simulink model "tav1"  (R2025b)
settings: Solver=FixedStepAuto  StartTime=0.0  StopTime=20  FixedStep=0.005  RelTol=1e-3
libraries: robotmaniplib x12
settings Model: Creator=giuli  LastModifiedBy=Andrea

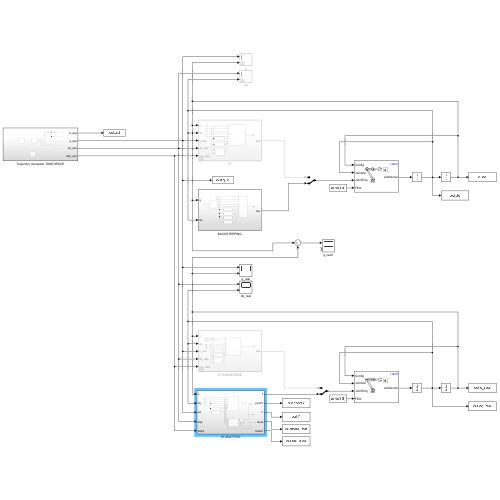
[thumbnail: Simulink's stored preview of the top-level diagram]
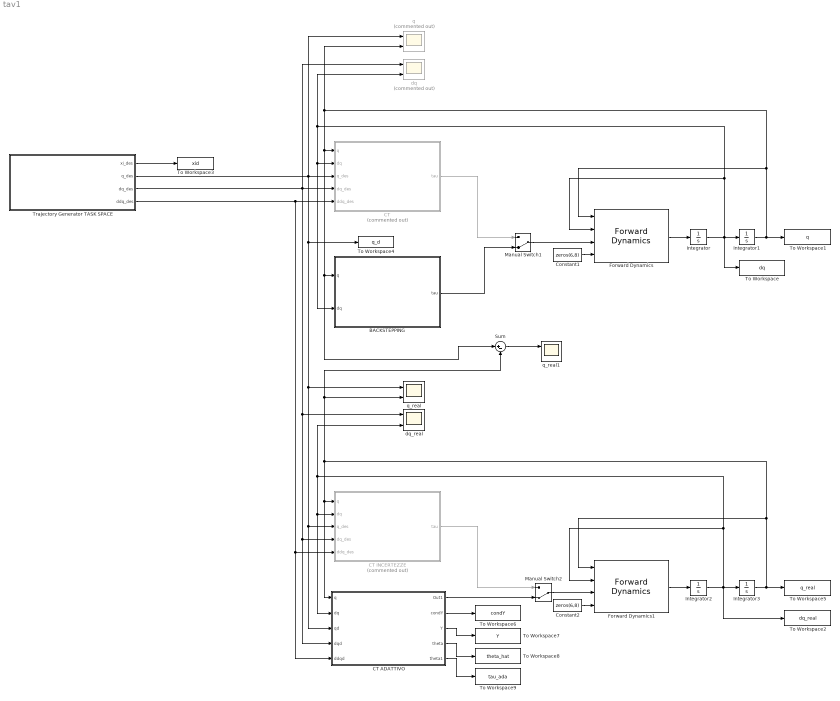
== system tav1 ==
  BACKSTEPPING : Subsystem
  CT : Subsystem  Commented=on
  CT ADATTIVO : Subsystem
  CT INCERTEZZE : Subsystem  Commented=on
  Constant1 : Constant  Value=zeros(6,8)
  Constant2 : Constant  Value=zeros(6,8)
  Forward Dynamics : robotmaniplib/Forward Dynamics  RigidBodyTree=robot  SimulateUsing=Interpreted execution
  Forward Dynamics1 : robotmaniplib/Forward Dynamics  RigidBodyTree=robot  SimulateUsing=Interpreted execution
  Integrator{,1..3} (4 alike) : Integrator  InitialCondition=zeros(6,1)
  Manual Switch1 : ManualSwitch  CurrentSetting=0
  Manual Switch2 : ManualSwitch  CurrentSetting=0
  Sum : Sum  Inputs=|+-
  To Workspace : ToWorkspace  VariableName=dq  SaveFormat=Timeseries  SampleTime=-1
  To Workspace1 : ToWorkspace  VariableName=q  SaveFormat=Timeseries  SampleTime=-1
  To Workspace2 : ToWorkspace  VariableName=dq_real  SaveFormat=Timeseries  SampleTime=-1
  To Workspace3 : ToWorkspace  VariableName=xid  SaveFormat=Timeseries  SampleTime=-1
  To Workspace4 : ToWorkspace  VariableName=q_d  SaveFormat=Timeseries  SampleTime=-1
  To Workspace5 : ToWorkspace  VariableName=q_real  SaveFormat=Timeseries  SampleTime=-1
  To Workspace6 : ToWorkspace  VariableName=condY  SaveFormat=Timeseries  SampleTime=-1
  To Workspace7 : ToWorkspace  VariableName=Y  SaveFormat=Timeseries  SampleTime=-1
  To Workspace8 : ToWorkspace  VariableName=theta_hat  SaveFormat=Timeseries  SampleTime=-1
  To Workspace9 : ToWorkspace  VariableName=tau_ada  SaveFormat=Timeseries  SampleTime=-1
  Trajectory Generator TASK SPACE : Subsystem
  dq : Scope  Commented=on  NumInputPorts=2
      settings: ActiveDisplayYMinimum=-3.470657788298241  ActiveDisplayYMaximum=1.9321669789401574  DataLoggingVariableName=ScopeData3
  dq_real : Scope  NumInputPorts=2
      settings: ActiveDisplayYMinimum=-6.9956803781599319  ActiveDisplayYMaximum=9.2235365390379016  DataLoggingVariableName=ScopeData2
  q : Scope  Commented=on  NumInputPorts=2
      settings: ActiveDisplayYMinimum=-2.5892485172575581  ActiveDisplayYMaximum=1.7379165019175062
  q_real : Scope  NumInputPorts=2
      settings: ActiveDisplayYMinimum=-6.9462044965016778  ActiveDisplayYMaximum=2.2220227218335191  DataLoggingVariableName=ScopeData4
  q_real1 : Scope  NumInputPorts=2
      settings: ActiveDisplayYMinimum=-0.19703612887750396  ActiveDisplayYMaximum=0.21289982446826508  DataLoggingVariableName=ScopeData5
  wires:
  Forward Dynamics/1 -> Integrator/1
  Integrator/1 -> To Workspace/1, Forward Dynamics/2, dq/2, BACKSTEPPING/2(dq), CT/2(dq), Integrator1/1
  Integrator1/1 -> q/2, Sum/1, BACKSTEPPING/1(q), CT/1(q), Forward Dynamics/1, To Workspace1/1
  Constant1/1 -> Forward Dynamics/4
  Trajectory Generator TASK SPACE/1(xi_des) -> To Workspace3/1
  Manual Switch1/1 -> Forward Dynamics/3
  CT/1(tau) -> Manual Switch1/1
  BACKSTEPPING/1(tau) -> Manual Switch1/2
  CT INCERTEZZE/1(tau) -> Manual Switch2/1
  Integrator2/1 -> Integrator3/1, dq_real/2, CT INCERTEZZE/2(dq), CT ADATTIVO/2(dq), Forward Dynamics1/2, To Workspace2/1
  Constant2/1 -> Forward Dynamics1/4
  Sum/1 -> q_real1/1
  Trajectory Generator TASK SPACE/4(ddq_des) -> CT ADATTIVO/5(ddqd), CT INCERTEZZE/5(ddq_des), CT/5(ddq_des)
  Trajectory Generator TASK SPACE/2(q_des) -> q/1, CT/3(q_des), CT ADATTIVO/3(qd), CT INCERTEZZE/3(q_des), q_real/1, To Workspace4/1
  Trajectory Generator TASK SPACE/3(dq_des) -> dq/1, CT/4(dq_des), CT ADATTIVO/4(dqd), CT INCERTEZZE/4(dq_des), dq_real/1
  Forward Dynamics1/1 -> Integrator2/1
  Manual Switch2/1 -> Forward Dynamics1/3
  Integrator3/1 -> To Workspace5/1, q_real/2, Sum/2, CT ADATTIVO/1(q), CT INCERTEZZE/1(q), Forward Dynamics1/1
  CT ADATTIVO/1(Out1) -> Manual Switch2/2
  CT ADATTIVO/2(condY) -> To Workspace6/1
  CT ADATTIVO/3(Y) -> To Workspace7/1
  CT ADATTIVO/4(theta) -> To Workspace8/1
  CT ADATTIVO/5(theta1) -> To Workspace9/1

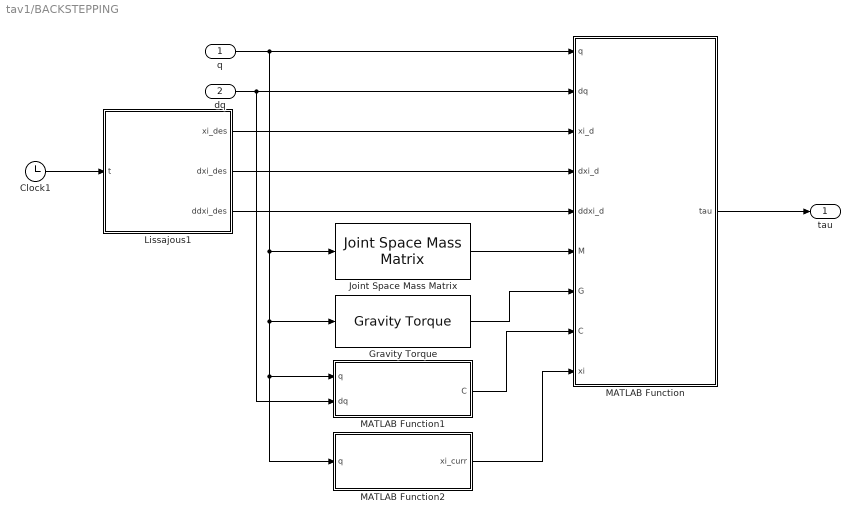
== system tav1/BACKSTEPPING ==
  q : Inport
  dq : Inport  Port=2
  Clock1 : Clock
  Gravity Torque : robotmaniplib/Gravity Torque  RigidBodyTree=robot  SimulateUsing=Interpreted execution
  Joint Space Mass Matrix : robotmaniplib/Joint Space Mass Matrix  RigidBodyTree=robot  SimulateUsing=Interpreted execution
  Lissajous1 : MATLAB Function  TreatAsAtomicUnit=on
  MATLAB Function : MATLAB Function  TreatAsAtomicUnit=on
  MATLAB Function1 : MATLAB Function  TreatAsAtomicUnit=on
  MATLAB Function2 : MATLAB Function  TreatAsAtomicUnit=on
  tau : Outport
  wires:
  dq/1 -> MATLAB Function1/2(dq), MATLAB Function/2(dq)
  q/1 -> Joint Space Mass Matrix/1, Gravity Torque/1, MATLAB Function2/1(q), MATLAB Function1/1(q), MATLAB Function/1(q)
  Joint Space Mass Matrix/1 -> MATLAB Function/6(M)
  Gravity Torque/1 -> MATLAB Function/7(G)
  MATLAB Function/1(tau) -> tau/1
  Clock1/1 -> Lissajous1/1(t)
  Lissajous1/1(xi_des) -> MATLAB Function/3(xi_d)
  Lissajous1/2(dxi_des) -> MATLAB Function/4(dxi_d)
  Lissajous1/3(ddxi_des) -> MATLAB Function/5(ddxi_d)
  MATLAB Function2/1(xi_curr) -> MATLAB Function/9(xi)
  MATLAB Function1/1(C) -> MATLAB Function/8(C)

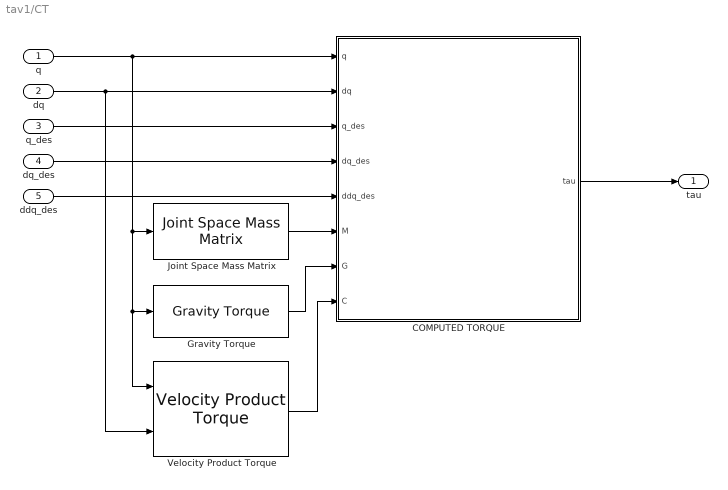
== system tav1/CT ==
  q : Inport
  dq : Inport  Port=2
  q_des : Inport  Port=3
  dq_des : Inport  Port=4
  ddq_des : Inport  Port=5
  COMPUTED TORQUE : MATLAB Function  TreatAsAtomicUnit=on
  Gravity Torque : robotmaniplib/Gravity Torque  RigidBodyTree=robot  SimulateUsing=Interpreted execution
  Joint Space Mass Matrix : robotmaniplib/Joint Space Mass Matrix  RigidBodyTree=robot  SimulateUsing=Interpreted execution
  Velocity Product Torque : robotmaniplib/Velocity Product Torque  RigidBodyTree=robot  SimulateUsing=Interpreted execution
  tau : Outport
  wires:
  COMPUTED TORQUE/1(tau) -> tau/1
  q_des/1 -> COMPUTED TORQUE/3(q_des)
  dq/1 -> Velocity Product Torque/2, COMPUTED TORQUE/2(dq)
  q/1 -> Velocity Product Torque/1, Gravity Torque/1, Joint Space Mass Matrix/1, COMPUTED TORQUE/1(q)
  dq_des/1 -> COMPUTED TORQUE/4(dq_des)
  ddq_des/1 -> COMPUTED TORQUE/5(ddq_des)
  Joint Space Mass Matrix/1 -> COMPUTED TORQUE/6(M)
  Gravity Torque/1 -> COMPUTED TORQUE/7(G)
  Velocity Product Torque/1 -> COMPUTED TORQUE/8(C)

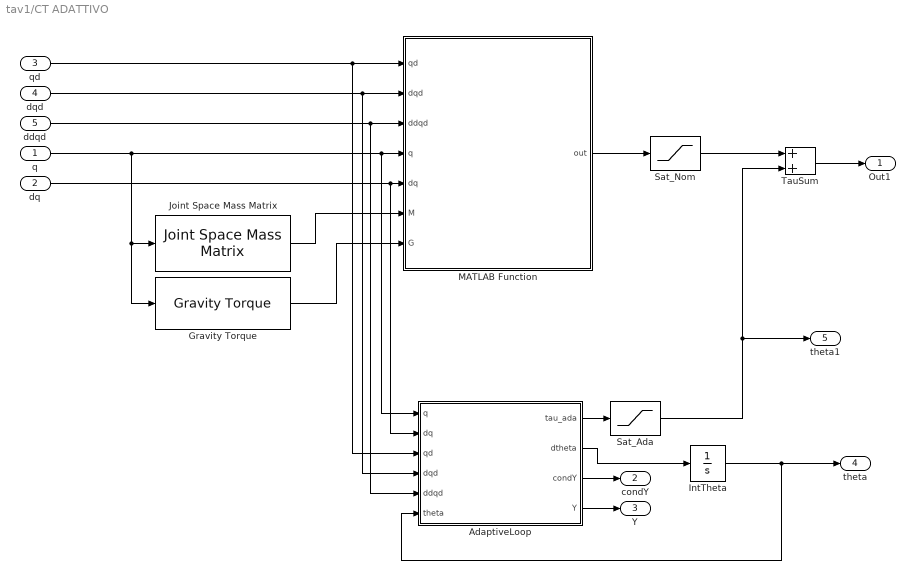
== system tav1/CT ADATTIVO ==
  q : Inport
  dq : Inport  Port=2
  qd : Inport  Port=3
  dqd : Inport  Port=4
  ddqd : Inport  Port=5
  AdaptiveLoop : MATLAB Function  TreatAsAtomicUnit=on
  Gravity Torque : robotmaniplib/Gravity Torque  RigidBodyTree=robot_real  SimulateUsing=Interpreted execution
  IntTheta : Integrator  InitialCondition=[0;0;0;0;0;0;0;0;0;0;0;0;0;0;0;0;0;0;0;0;0;0;0;0;0;0;0;0;0;0;0;0;0;0;0;0;0;0;0;0;0;0]
  Joint Space Mass Matrix : robotmaniplib/Joint Space Mass Matrix  RigidBodyTree=robot_real  SimulateUsing=Interpreted execution
  MATLAB Function : MATLAB Function  TreatAsAtomicUnit=on
  Sat_Ada : Saturate  UpperLimit=100  LowerLimit=-100
  Sat_Nom : Saturate  UpperLimit=100  LowerLimit=-100
  TauSum : Sum
  Out1 : Outport
  condY : Outport  Port=2
  Y : Outport  Port=3
  theta : Outport  Port=4
  theta1 : Outport  Port=5
  wires:
  q/1 -> AdaptiveLoop/1(q), MATLAB Function/4(q), Joint Space Mass Matrix/1, Gravity Torque/1
  Sat_Nom/1 -> TauSum/1
  qd/1 -> MATLAB Function/1(qd), AdaptiveLoop/3(qd)
  TauSum/1 -> Out1/1
  ddqd/1 -> MATLAB Function/3(ddqd), AdaptiveLoop/5(ddqd)
  AdaptiveLoop/1(tau_ada) -> Sat_Ada/1
  AdaptiveLoop/2(dtheta) -> IntTheta/1
  dq/1 -> AdaptiveLoop/2(dq), MATLAB Function/5(dq)
  Sat_Ada/1 -> TauSum/2, theta1/1
  IntTheta/1 -> theta/1, AdaptiveLoop/6(theta)
  dqd/1 -> MATLAB Function/2(dqd), AdaptiveLoop/4(dqd)
  MATLAB Function/1(out) -> Sat_Nom/1
  Gravity Torque/1 -> MATLAB Function/7(G)
  Joint Space Mass Matrix/1 -> MATLAB Function/6(M)
  AdaptiveLoop/3(condY) -> condY/1
  AdaptiveLoop/4(Y) -> Y/1

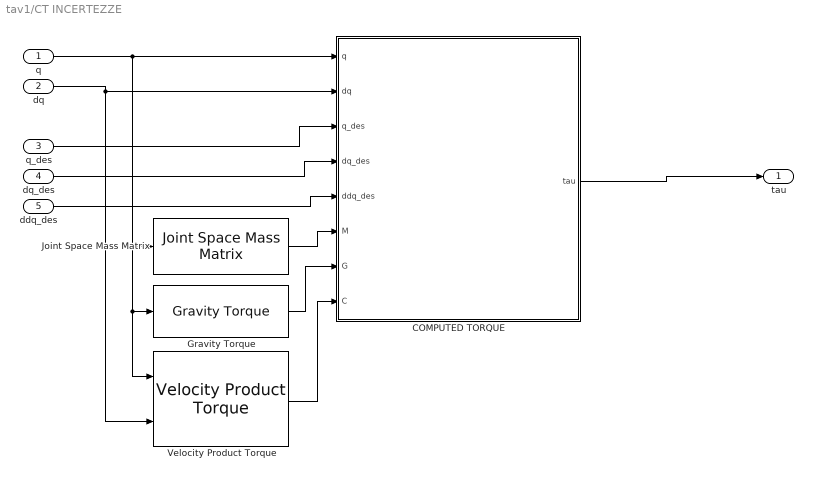
== system tav1/CT INCERTEZZE ==
  q : Inport
  dq : Inport  Port=2
  q_des : Inport  Port=3
  dq_des : Inport  Port=4
  ddq_des : Inport  Port=5
  COMPUTED TORQUE : MATLAB Function  TreatAsAtomicUnit=on
  Gravity Torque : robotmaniplib/Gravity Torque  RigidBodyTree=robot_real  SimulateUsing=Interpreted execution
  Joint Space Mass Matrix : robotmaniplib/Joint Space Mass Matrix  RigidBodyTree=robot_real  SimulateUsing=Interpreted execution
  Velocity Product Torque : robotmaniplib/Velocity Product Torque  RigidBodyTree=robot_real  SimulateUsing=Interpreted execution
  tau : Outport
  wires:
  COMPUTED TORQUE/1(tau) -> tau/1
  q_des/1 -> COMPUTED TORQUE/3(q_des)
  dq/1 -> Velocity Product Torque/2, COMPUTED TORQUE/2(dq)
  q/1 -> Velocity Product Torque/1, Gravity Torque/1, Joint Space Mass Matrix/1, COMPUTED TORQUE/1(q)
  dq_des/1 -> COMPUTED TORQUE/4(dq_des)
  ddq_des/1 -> COMPUTED TORQUE/5(ddq_des)
  Joint Space Mass Matrix/1 -> COMPUTED TORQUE/6(M)
  Gravity Torque/1 -> COMPUTED TORQUE/7(G)
  Velocity Product Torque/1 -> COMPUTED TORQUE/8(C)

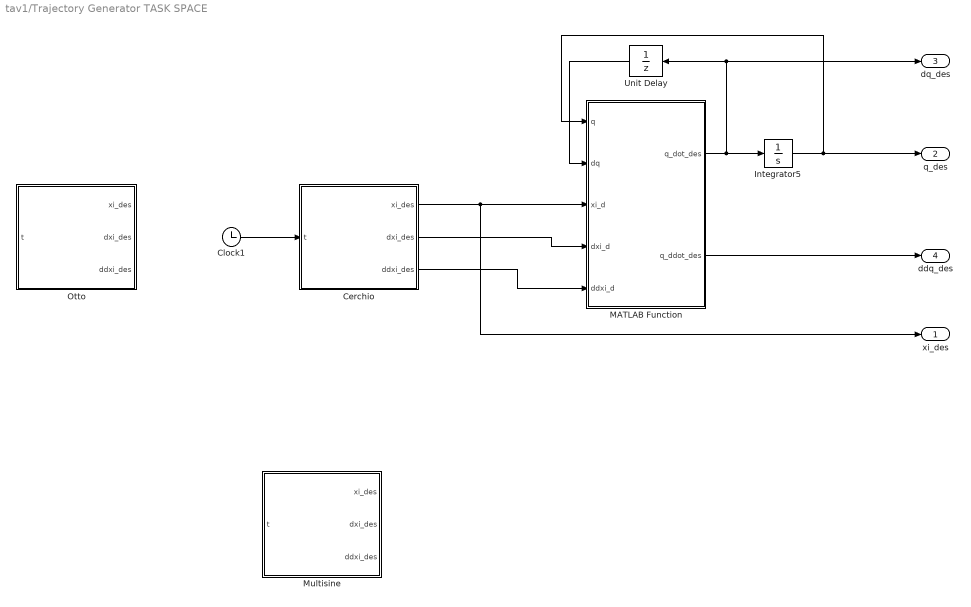
== system tav1/Trajectory Generator TASK SPACE ==
  Cerchio : MATLAB Function  TreatAsAtomicUnit=on
  Clock1 : Clock
  Integrator5 : Integrator  InitialCondition=[0;1.3052;-0.0773;-0;-1.2279;0]
  MATLAB Function : MATLAB Function  TreatAsAtomicUnit=on
  Multisine : MATLAB Function  TreatAsAtomicUnit=on
  Otto : MATLAB Function  TreatAsAtomicUnit=on
  Unit Delay : UnitDelay  InitialCondition=[0; 0.1; -0.073; 0; 0.2736; 0]  SampleTime=-1  HasFrameUpgradeWarning=on
  xi_des : Outport
  q_des : Outport  Port=2
  dq_des : Outport  Port=3
  ddq_des : Outport  Port=4
  wires:
  Unit Delay/1 -> MATLAB Function/2(dq)
  MATLAB Function/1(q_dot_des) -> Integrator5/1, Unit Delay/1, dq_des/1
  MATLAB Function/2(q_ddot_des) -> ddq_des/1
  Integrator5/1 -> q_des/1, MATLAB Function/1(q)
  Clock1/1 -> Cerchio/1(t)
  Cerchio/1(xi_des) -> xi_des/1, MATLAB Function/3(xi_d)
  Cerchio/2(dxi_des) -> MATLAB Function/4(dxi_d)
  Cerchio/3(ddxi_des) -> MATLAB Function/5(ddxi_d)

== matlab function tav1/CT INCERTEZZE/COMPUTED TORQUE ==
  data: q input; dq input; q_des input; dq_des input; ddq_des input; tau output; M input; G input; C input
function tau = computed_torque(q, dq, q_des, dq_des, ddq_des, M, G, C)

% control parameters
kp = 5;
kv = 2;

% error computation
e = q_des - q;
de = dq_des - dq;

tau = M*(ddq_des + kv*de + kp*e) + C + G;

== matlab function tav1/CT ADATTIVO/MATLAB Function ==
  data: qd input; out output; dqd input; ddqd input; q input; dq input; M input; G input
function out = fcn(qd,dqd,ddqd,q,dq, M, G)
    coder.extrinsic('velocityProduct');
    coder.extrinsic('evalin');
    
    % Recupero robot e nome end-effector dal base workspace
    robot = evalin('base','robot_real');                  % rigidBodyTree abbIrb120

    Kd   = 20*eye(6);
    Lam  = 2*eye(6);
    e    = qd-q;  de = dqd-dq;
    dqr  = ddqd + Lam*de;
    ar   = dqr  + Kd*(de+Lam*e);
    VP = zeros(6,1);  
    VP  = velocityProduct(robot, q, dq);   

    out = zeros(6,1);  
    out = M * ar + VP + G;

end

== matlab function tav1/Trajectory Generator TASK SPACE/Otto ==
  data: t input; xi_des output; dxi_des output; ddxi_des output
function [xi_des, dxi_des, ddxi_des] = traj_otto(t)
% FIGURA A OTTO (Lissajous 2:1)
%
% Punto iniziale IDENTICO al cerchio originale (lissajous.m):
%   t=0 -> xi = [0.50; 0.00; 0.10; 0; 0; 0]
%          dxi = [0; R*w; 0; 0; 0; 0] = [0; 0.30; 0; 0; 0; 0]
%
% Raccordo posizione:
%   x(t) = x0 + Rx * sin(2*w*t + pi/2)   →  x(0) = x0 + Rx = 0.50  ✓
%   y(t) = y0 + Ry * sin(w*t)             →  y(0) = 0               ✓
%   z(t) = z0                             →  z(0) = 0.10             ✓
%
% Raccordo velocità:
%   dx(0) = 2*w*Rx*cos(pi/2) = 0          ✓  (cerchio: dx(0) = 0)
%   dy(0) = w*Ry              = 0.30       →  Ry = 0.15 = R          ✓
%
% => Rx = Ry = R = 0.15, w = 2 (invariati dal cerchio)

%% Parametri (coerenti con lissajous.m)
x0 = 0.35;
y0 = 0.00;
z0 = 0.10;
R  = 0.15;
w  = 2.0;

%% Orientazione variabile (nulla a t=0, eccita Coriolis)
A_roll  = 0.10;   % ampiezza roll  [rad]
A_pitch = 0.08;   % ampiezza pitch [rad]
w_o     = 0.7;    % freq incommensurabile con w  → PE
% uso sin() → valore nullo a t=0  ✓

%% --- POSIZIONE ---
p_des = [ x0 + R * sin(2*w*t + pi/2);
          y0 + R * sin(w*t);
          z0                          ];

%% --- VELOCITÀ ---
dp_des = [ 2*w*R * cos(2*w*t + pi/2);
           w*R   * cos(w*t);
           0                          ];

%% --- ACCELERAZIONE ---
ddp_des = [ -4*w^2*R * sin(2*w*t + pi/2);
            -w^2*R   * sin(w*t);
             0                            ];

%% --- ORIENTAZIONE (sin -> 0 a t=0) ---
roll  = A_roll  * sin(w_o * t);
pitch = A_pitch * sin(w_o * t);
yaw   = 0;

o_des   = [roll; pitch; yaw];
do_des  = [ A_roll*w_o  * cos(w_o*t);
            A_pitch*w_o * cos(w_o*t);
            0                        ];
ddo_des = [-A_roll*w_o^2  * sin(w_o*t);
           -A_pitch*w_o^2 * sin(w_o*t);
            0                          ];

%% --- ROTAZIONE ZYX ---
cr = cos(roll);  sr = sin(roll);
cp = cos(pitch); sp = sin(pitch);
cy = cos(yaw);   sy = sin(yaw);
R_mat = [ cy*cp,  cy*sp*sr - sy*cr,  cy*sp*cr + sy*sr;
          sy*cp,  sy*sp*sr + cy*cr,  sy*sp*cr - cy*sr;
         -sp,     cp*sr,             cp*cr            ];
T = eye(4);  T(1:3,1:3) = R_mat;  T(1:3,4) = p_des;

%% --- OUTPUT ---
xi_des   = [p_des;   o_des  ];
dxi_des  = [dp_des;  do_des ];
ddxi_des = [ddp_des; ddo_des];
end

== matlab function tav1/Trajectory Generator TASK SPACE/Multisine ==
  data: t input; xi_des output; dxi_des output; ddxi_des output
function [xi_des, dxi_des, ddxi_des] = traj_multisine(t)
% MULTI-SINE 3D — MASSIMA ECCITAZIONE PERSISTENTE
%
% Punto iniziale IDENTICO al cerchio originale (lissajous.m):
%   t=0 -> xi = [0.50; 0.00; 0.10; 0; 0; 0]
%          dxi = [0; 0.30; 0; 0; 0; 0]
%
% Strategia di raccordo:
%   Per ogni asse si usa una somma di coseni sfasati in modo che:
%     p(0)  = p0_cerchio   →  offset + sum(Ak*cos(phik))   = valore target
%     dp(0) = dp0_cerchio  →  -sum(Ak*wk*sin(phik))        = valore target
%
%   Sul piano x: p(0)=0.50, dp(0)=0  → offset=0.50, tutti sin(wk*t) puri
%                (sin(0)=0, d/dt sin(wk*t)|t=0 = wk ≠ 0 → serve correzione)
%
%   Soluzione pratica: usare cos(wk*t - pi/2) = sin(wk*t)  su y
%   e cos(wk*t) su x con offset calibrato.
%
%   x(t) = x0 + R + sum_k[ Axk*(cos(wxk*t) - 1) ]
%          → x(0) = x0 + R = 0.50  (i termini (cos-1) si annullano)  ✓
%          → dx(0)= -sum(Axk*wxk*sin(0)) = 0                          ✓
%
%   y(t) = y0 + sum_k[ Ayk*sin(wyk*t) ]
%          → y(0) = 0                                                  ✓
%          → dy(0)= sum(Ayk*wyk)  → scelti Ayk e wyk st sum = R*w=0.30 ✓
%
%   z(t) = z0 + sum_k[ Azk*(cos(wzk*t) - 1) ]
%          → z(0) = z0 = 0.10                                          ✓
%          → dz(0)= 0                                                  ✓
%
%   Orientazione: tutte sin() → nulle a t=0                            ✓

%% Parametri base (dal cerchio)
x0 = 0.35;
y0 = 0.00;
z0 = 0.10;
R  = 0.15;
w  = 2.0;

%% Frequenze incommensurabili [rad/s]  1 : sqrt(2) : sqrt(3)
w1 = 1.0000;
w2 = 1.4142;   % sqrt(2)
w3 = 1.7321;   % sqrt(3)

%% Ampiezze asse x  (cos -> dc offset calibrato)
Ax = [0.08, 0.05, 0.04];
wx = [w1,   w2,   w3  ];
% x(0) = x0 + R + sum(Ax*(cos(0)-1)) = x0 + R + 0 = 0.50  ✓
% dx(0) = 0  ✓

%% Ampiezze asse y  (sin)
% Vincolo: sum(Ayk*wyk) = R*w = 0.15*2 = 0.30
% Scelta:  Ay1*w_y1 + Ay2*w_y2 + Ay3*w_y3 = 0.30
%   0.10*1.0 + 0.10*1.4142 + 0.10*0.5858 ≈ 0.10+0.1414+0.0586 = 0.30  ✓
Ay = [0.10,  0.10,   0.10  ];
wy = [w1,    w2,     0.5858];   % 0.5858 = 2 - sqrt(2)

%% Ampiezze asse z  (cos -> offset)
Az = [0.04, 0.02, 0.01];
wz = [w2,   w3,   w1*0.5];
% z(0) = z0 + sum(Az*(1-1)) = z0  ✓

%% --- POSIZIONE ---
px = x0 + R + sum(Ax .* (cos(wx*t) - 1));
py = y0      + sum(Ay .*  sin(wy*t)     );
pz = z0      + sum(Az .* (cos(wz*t) - 1));
p_des = [px; py; pz];

%% --- VELOCITÀ ---
dpx = -sum(Ax .* wx .* sin(wx*t));
dpy =  sum(Ay .* wy .* cos(wy*t));
dpz = -sum(Az .* wz .* sin(wz*t));
dp_des = [dpx; dpy; dpz];

%% --- ACCELERAZIONE ---
ddpx = -sum(Ax .* wx.^2 .* cos(wx*t));
ddpy = -sum(Ay .* wy.^2 .* sin(wy*t));
ddpz = -sum(Az .* wz.^2 .* cos(wz*t));
ddp_des = [ddpx; ddpy; ddpz];

%% --- ORIENTAZIONE (sin -> 0 a t=0) ---
w_o = [0.6, 0.9, 1.2];
Ar  = [0.08, 0.04, 0.02];
Ap  = [0.06, 0.03, 0.02];
Ay2 = [0.05, 0.03, 0.01];

roll  = sum(Ar  .* sin(w_o*t));
pitch = sum(Ap  .* sin(w_o*t));
yaw   = sum(Ay2 .* sin(w_o*t));

o_des   = [roll; pitch; yaw];
do_des  = [ sum(Ar  .* w_o .* cos(w_o*t));
            sum(Ap  .* w_o .* cos(w_o*t));
            sum(Ay2 .* w_o .* cos(w_o*t)) ];
ddo_des = [-sum(Ar  .* w_o.^2 .* sin(w_o*t));
           -sum(Ap  .* w_o.^2 .* sin(w_o*t));
           -sum(Ay2 .* w_o.^2 .* sin(w_o*t)) ];

%% --- ROTAZIONE ZYX ---
cr = cos(roll);  sr = sin(roll);
cp = cos(pitch); sp = sin(pitch);
cy = cos(yaw);   sy = sin(yaw);
R_mat = [ cy*cp,  cy*sp*sr - sy*cr,  cy*sp*cr + sy*sr;
          sy*cp,  sy*sp*sr + cy*cr,  sy*sp*cr - cy*sr;
         -sp,     cp*sr,             cp*cr            ];
T = eye(4);  T(1:3,1:3) = R_mat;  T(1:3,4) = p_des;

%% --- OUTPUT ---
xi_des   = [p_des;   o_des  ];
dxi_des  = [dp_des;  do_des ];
ddxi_des = [ddp_des; ddo_des];
end

== matlab function tav1/CT ADATTIVO/AdaptiveLoop ==
  data: q input; tau_ada output; dq input; qd input; dqd input; ddqd input; theta input; dtheta output; condY output; Y output
function [tau_ada, dtheta, condY, Y] = fcn(q,dq,qd,dqd,ddqd,theta)

tau_ada = zeros(6,1);
dtheta  = zeros(42,1);
Lam   = 2  * eye(6);   
Gam   = 0.3  * eye(42);  
sigma = 0.05;            
eps_s = 0.05;             
e   = qd  - q;
de  = dqd - dq;
dqr = ddqd + Lam*de;
sr  = de   + Lam*e;

Y = zeros(6,42);
for i = 1:6
    b = int32((i-1)*7);
    Y(i,b+1) = dqr(i);
    Y(i,b+2) = dq(i)^2 * tanh(sr(i)/eps_s);
    Y(i,b+3) = dq(i);
    Y(i,b+4) = q(i);
    Y(i,b+5) = sin(q(i));
    Y(i,b+6) = cos(q(i));
    Y(i,b+7) = tanh(dq(i)/eps_s);
end

condY = cond(Y);

tau_ada = Y * theta;
dtheta  = Gam*(Y'*sr) - sigma*theta;

== matlab function tav1/BACKSTEPPING/Lissajous1 ==
  data: t input; xi_des output; dxi_des output; ddxi_des output
function [xi_des, dxi_des, ddxi_des] = lissajous(t)
% CIRCLE TRAJECTORY WITH ORIENTATION (6D task)
% xi = [x; y; z; roll; pitch; yaw]

%% Position parameters
x0 = 0.35;
y0 = 0;
z0 = 0.10;
R  = 0.15;
w  = 2;

%% Orientation (constant)
roll  = 0;
pitch = 0;
yaw   = 0;

%% Desired position (3x1)
p_des = [ x0 + R*cos(w*t);
          y0 + R*sin(w*t);
          z0 ];

%% Desired velocity (3x1)
dp_des = [ -R*w*sin(w*t);
            R*w*cos(w*t);
            0 ];

%% Desired acceleration (3x1)
ddp_des = [ -R*w^2*cos(w*t);
            -R*w^2*sin(w*t);
             0 ];

%% Orientation (constant) → 0 velocity, 0 acceleration
o_des    = [roll; pitch; yaw];
do_des   = [0; 0; 0];
ddo_des  = [0; 0; 0];

%% Rotation matrix (ZYX: yaw-pitch-roll)
cr = cos(roll);  sr = sin(roll);
cp = cos(pitch); sp = sin(pitch);
cy = cos(yaw);   sy = sin(yaw);

R = [ cy*cp,  cy*sp*sr - sy*cr,  cy*sp*cr + sy*sr;
      sy*cp,  sy*sp*sr + cy*cr,  sy*sp*cr - cy*sr;
      -sp,    cp*sr,             cp*cr ];

%% Homogeneous transform
T = eye(4);
T(1:3,1:3) = R;
T(1:3,4)   = [p_des(1); p_des(2); p_des(3)];


%% Final 6x1 outputs
xi_des   = [p_des;  o_des];
dxi_des  = [dp_des; do_des];
ddxi_des = [ddp_des; ddo_des];

end

== matlab function tav1/BACKSTEPPING/MATLAB Function ==
  settings: updateMethod=DISCRETE
  data: q input; tau output; dq input; xi_d input; dxi_d input; ddxi_d input; M input; G input; C input; xi input
function tau = fcn(q, dq, xi_d, dxi_d, ddxi_d, M, G, C, xi)

% Funzioni extrinsic (non generabili) dichiarate per il coder
coder.extrinsic('geometricJacobian');
coder.extrinsic('velocityProduct');
coder.extrinsic('evalin');

% Recupero robot e nome end-effector dal base workspace
robot = evalin('base','robot');                  % rigidBodyTree abbIrb120
ee    = evalin('base','robot.Bodies{end}.Name'); % "tool0" nel tuo caso

J   = zeros(6,6);
J2   = zeros(6,6);
J_dot  = zeros(6,6);

% 1) Jacobiano J(q)
Jtmp = geometricJacobian(robot, q, ee);   % mxArray 6x6
J(:,:) = double(Jtmp);                   % conversione a double 6x6
J = [J(4:6,:); J(1:3,:)];

% ---------------------------------------------------------
% 2) Derivata numerica Jdot lungo dq
eps = 1e-6;
q2  = q + eps * dq;

Jtmp2 = geometricJacobian(robot, q2, ee);
J2(:,:) = double(Jtmp2);
J2 = [J2(4:6,:); J2(1:3,:)];

J_dot(:,:) = (J2 - J) / eps;

% opzionale: se le velocità sono quasi nulle, azzero Jdot per evitare rumore
if norm(dq) < 1e-4
    J_dot(:,:) = zeros(6,6);
end

% gains
lambda = 20;
kd = 0.30;

% kinematics
e = xi_d - xi;

pinv_J = pinv(J);

dq_r = pinv_J * (dxi_d + lambda*e);
ddq_r = pinv_J * (ddxi_d + lambda*dxi_d - lambda*J*dq) - pinv_J * J_dot * pinv_J * (dxi_d + lambda*e);

s = dq_r - dq;

tau = M*ddq_r + C * dq_r + G + kd*s + J'*e;

== matlab function tav1/Trajectory Generator TASK SPACE/MATLAB Function ==
  data: q_dot_des output; q input; dq input; xi_d input; dxi_d input; ddxi_d input; q_ddot_des output
function [q_dot_des,q_ddot_des]   = ee2joint_kin(q, dq, xi_d, dxi_d, ddxi_d)
% ee2joint_kin
% Data la traiettoria desiderata dell'end-effector (xi_d, dxi_d, ddxi_d),
% calcola le velocità e accelerazioni di giunto desiderate (q_dot_des, q_ddot_des)
% usando inversione cinematica differenziale 6D.
%
% INPUT:
%   q       : 6x1 configurazione attuale desiderata (q_d)
%   dq      : 6x1 velocità giunti desiderata corrente (q_dot_d)
%   xi_d    : 6x1 [x;y;z;roll;pitch;yaw] desiderati
%   dxi_d   : 6x1 velocità task desiderata
%   ddxi_d  : 6x1 accelerazione task desiderata
%
% OUTPUT:
%   q_dot_des  : 6x1 velocità giunti desiderata
%   q_ddot_des : 6x1 accelerazione giunti desiderata

% ---------------------------------------------------------
% Preallocazioni con dimensioni fisse per Simulink
q_dot_des  = zeros(6,1);
q_ddot_des = zeros(6,1);

J   = zeros(6,6);
J2   = zeros(6,6);
dJ  = zeros(6,6);

% ---------------------------------------------------------
% Funzioni extrinsic (non generabili) dichiarate per il coder
%  
coder.extrinsic('geometricJacobian');
coder.extrinsic('getTransform','tform2trvec','tform2eul');
coder.extrinsic('evalin');

% Recupero robot e nome end-effector dal base workspace
robot = evalin('base','robot');                  % rigidBodyTree abbIrb120
ee    = evalin('base','robot.Bodies{end}.Name'); % "tool0" nel tuo caso

% ---------------------------------------------------------
% 1) Jacobiano J(q)
Jtmp = geometricJacobian(robot, q, ee);   % mxArray 6x6
J(:,:) = double(Jtmp);                   % conversione a double 6x6
J = [J(4:6,:); J(1:3,:)];

% ---------------------------------------------------------
% 2) Derivata numerica Jdot lungo dq
eps = 1e-6;
q2  = q + eps * dq;

Jtmp2 = geometricJacobian(robot, q2, ee);
J2(:,:) = double(Jtmp2);
J2 = [J2(4:6,:); J2(1:3,:)];

dJ(:,:) = (J2 - J) / eps;

% opzionale: se le velocità sono quasi nulle, azzero Jdot per evitare rumore
if norm(dq) < 1e-4
    dJ(:,:) = zeros(6,6);
end

% ---------------------------------------------------------
% 4) Calcolo q_dot_des dalla velocità desiderata dxi_d
q_dot_des = pinv(J) * dxi_d;    % 6x1

% ---------------------------------------------------------
% 5) Calcolo q_ddot_des dalla accelerazione desiderata ddxi_d
%    usando: ddxi_d = J*ddq_d + Jdot*dq_d
%    => ddq_d = J# (ddxi_d - Jdot*dq_d)
q_ddot_des = pinv(J) * (ddxi_d - dJ * dq);


end

== matlab function tav1/CT/COMPUTED TORQUE ==
  data: q input; dq input; q_des input; dq_des input; ddq_des input; tau output; M input; G input; C input
function tau = computed_torque(q, dq, q_des, dq_des, ddq_des, M, G, C)

% control parameters
kp = 5;
kv = 2;

% error computation
e = q_des - q;
de = dq_des - dq;

tau = M*(ddq_des + kv*de + kp*e) + C + G;

== matlab function tav1/Trajectory Generator TASK SPACE/Cerchio ==
  data: t input; xi_des output; dxi_des output; ddxi_des output
function [xi_des, dxi_des, ddxi_des] = traj_cerchio(t)
% CIRCLE TRAJECTORY WITH ORIENTATION (6D task)
% xi = [x; y; z; roll; pitch; yaw]

%% Position parameters
x0 = 0.35;
y0 = 0;
z0 = 0.10;
R  = 0.15;
w  = 2;

%% Orientation (constant)
roll  = 0;
pitch = 0;
yaw   = 0;

%% Desired position (3x1)
p_des = [ x0 + R*cos(w*t);
          y0 + R*sin(w*t);
          z0 ];

%% Desired velocity (3x1)
dp_des = [ -R*w*sin(w*t);
            R*w*cos(w*t);
            0 ];

%% Desired acceleration (3x1)
ddp_des = [ -R*w^2*cos(w*t);
            -R*w^2*sin(w*t);
             0 ];

%% Orientation (constant) → 0 velocity, 0 acceleration
o_des    = [roll; pitch; yaw];
do_des   = [0; 0; 0];
ddo_des  = [0; 0; 0];

%% Rotation matrix (ZYX: yaw-pitch-roll)
cr = cos(roll);  sr = sin(roll);
cp = cos(pitch); sp = sin(pitch);
cy = cos(yaw);   sy = sin(yaw);

R = [ cy*cp,  cy*sp*sr - sy*cr,  cy*sp*cr + sy*sr;
      sy*cp,  sy*sp*sr + cy*cr,  sy*sp*cr - cy*sr;
      -sp,    cp*sr,             cp*cr ];

%% Homogeneous transform
T = eye(4);
T(1:3,1:3) = R;
T(1:3,4)   = [p_des(1); p_des(2); p_des(3)];


%% Final 6x1 outputs
xi_des   = [p_des;  o_des];
dxi_des  = [dp_des; do_des];
ddxi_des = [ddp_des; ddo_des];

end

== matlab function tav1/BACKSTEPPING/MATLAB Function1 ==
  settings: updateMethod=DISCRETE
  data: q input; C output; dq input
function C = get_C_norm(q, dq)
    coder.extrinsic('evalin');
    coder.extrinsic('massMatrix');

    robot = evalin('base','robot');

    n = length(q);
    C = zeros(n,n);
    
    eps = 1e-6;   
    
    % Derivate parziali di M rispetto a q_k
    dM = zeros(n,n,n);
    
    for k = 1:n
        qk_p = q;
        qk_m = q;
        qk_p(k) = qk_p(k) + eps;
        qk_m(k) = qk_m(k) - eps;
    
        Mp_tmp = massMatrix(robot, qk_p);
        Mp = zeros(6);
        Mp = double(Mp_tmp);
        Mm_tmp = massMatrix(robot, qk_m);
        Mm = zeros(6);
        Mm = double(Mm_tmp);
    
        dM(:,:,k) = (Mp - Mm) / (2*eps);
    end
    
    % Costruzione della matrice C
    for i = 1:n
        for j = 1:n
            for k = 1:n
                Gamma_ijk = 0.5 * (dM(i,j,k) + dM(i,k,j) - dM(j,k,i));
                C(i,j) = C(i,j) + Gamma_ijk * dq(k);
            end
        end
    end
end

== matlab function tav1/BACKSTEPPING/MATLAB Function2 ==
  settings: updateMethod=DISCRETE
  data: q input; xi_curr output
function xi_curr  = get_Xcurr_nom(q)
    coder.extrinsic('evalin');
    coder.extrinsic('getTransform');
    coder.extrinsic('tform2trvec');
    coder.extrinsic('tform2eul');

    robot = evalin('base','robot');
    ee = evalin('base','ee');

    T0 = getTransform(robot, q, ee);

    % Posa
    p0 = tform2trvec(T0)';

    % Orientamento in terna XYZ
    eul = tform2eul(T0, "XYZ")';

    xi_curr = zeros(6,1);
    xi_curr = [p0; eul];
end
